simulink model "dae_example"  (R2026b)
settings: Solver=VariableStepAuto  StopTime=20  MaxStep=0.4  AbsTol=1e-3  EnableMultiTasking=on
libraries: fl_lib x9, SimscapeFluids_lib x6, nesl_utility x1
CloseFcn:
  | try,close(h1_HydrostaticTransmissionWithSecondaryControl),end
  | clear h1_HydrostaticTransmissionWithSecondaryControl
  | 
  | clear simlog_HydrostaticTransmissionWithSecondaryControl tout
  | clear logsout_HydrostaticTransmissionWithSecondaryControl
settings Model: Creator=The MathWorks, Inc.  LastModifiedBy=grouleau
settings SolverCC: AutoScaleAbsTol=off
settings DataIOCC: DSMLogging=off  LimitDataPoints=on  MaxDataPoints=10000  ReturnWorkspaceOutputs=off  SaveFormat=Array  SignalLoggingName=logsout_HydrostaticTransmissionWithSecondaryControl
settings OptimizationCC: LifeSpan=inf  MemsetInitFltsAndDblsToZero=off  ReuseModelBlockBuffer=off
settings DebuggingCC: AllowSymbolicDim=off  ArithmeticOperatorsInVariantConditions=warning  PregeneratedLibrarySubsystemCodeDiagnostic=none  SFExecutionAtInitializationDiag=none  SFNoUnconditionalDefaultTransitionDiag=warning  SFUnexpectedBacktrackingDiag=warning  SaveWithParameterizedLinksMsg=none  SignalResolutionControl=TryResolveAllWithWarning  StateNameClashWarn=warning
settings HardwareCC: ProdEndianess=Unspecified  ProdHWDeviceType=32-bit Generic  ProdIntDivRoundTo=Undefined  ProdLargestAtomicFloat=None
settings ModelReferenceCC: PropagateSignalLabelsOutOfModel=off
settings SFSimCC: CustomCodeUndefinedFunction=UseInterfaceOnly  SimUseLocalCustomCode=off
settings RTWCC: DLArmComputeVersion=19.05  RTWUseLocalCustomCode=off
settings CodeAppCC: StateflowObjectComments=on
settings GRTTargetCC: CombineOutputUpdateFcns=off  GRTInterface=on  TargetFcnLib=ansi_tfl_tmw.mat  TargetLangStandard=C89/C90 (ANSI)
settings ConfigComp: CovExternalEMLEnable=off  CovSFcnEnable=off  CovSaveCumulativeToWorkspaceVar=on  CovSaveSingleToWorkspaceVar=on
settings SimscapeCC: SimscapeLogName=simlog_HydrostaticTransmissionWithSecondaryControl  SimscapeLogSimulationStatistics=on  SimscapeLogType=all  SimscapeUseEnergyAccounting=off

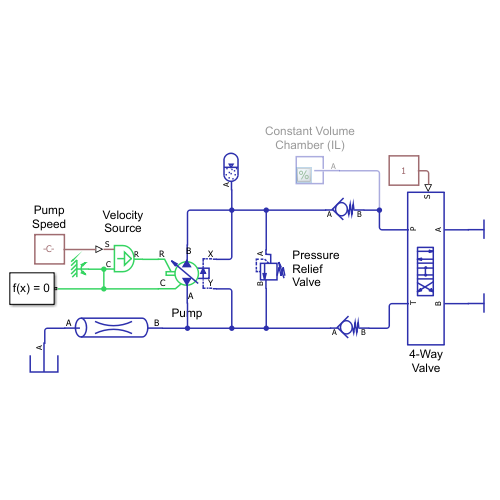
[thumbnail: Simulink's stored preview of the top-level diagram]
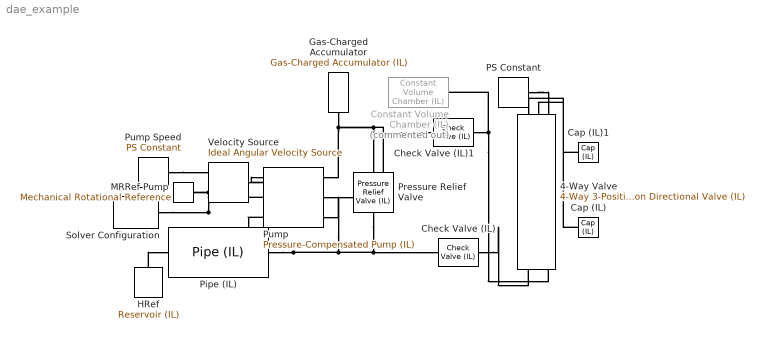
== system dae_example ==
  4-Way Valve : SimscapeFluids_lib/Isothermal Liquid/Valves & Orifices/Directional Control Valves/4-Way 3-Position Directional Valve (IL)  Tag=Factory Generic  open_orifices_pos=fluids.isothermal_liquid.valves_orifices.directional_control_valves.enum.directional_valve_open_orifices_pos_neg.PA_BT  open_orifices_neu=fluids.isothermal_liquid.valves_orifices.directional_control_valves.enum.directional_valve_open_orifices_neutral.PA_PB_AT_BT  open_orifices_neg=fluids.isothermal_liquid.valves_orifices.directional_control_valves.enum.directional_valve_open_orifices_pos_neg.PB_AT  neutral_assert_action=0  area_spec=1  valve_spec=1  del_S_max=5 mm  area_max=3.8 mm^2  del_S_TLU=[0, .00125, .0025, .00375, .005] m  valve_area_TLU="[  1e-12 4e-12 1e-05 1.02e-05 ] m^2"  del_S_vol_flow_TLU=[0, .00125, .0025, .00375, .005] m  p_diff_TLU="[  -5e+06 -2e+06 2e+06 5e+06 ] Pa"  vol_flow_TLU="[  -1e-12 -6e-14 6e+12 1e+11 ; -8e-08 -4e-08 4e+06 8e+06 ; -0.0025 -0.00103 0.001 0.0024 ; -0.00258 -0.001032 0.00106 0.00247 ; ] m^3/s"  p_diff_TLU_const=[-.1, .3, .5, .7] MPa  vol_flow_TLU_const=[-.0009, .0016, .002, .0024] m^3/s  area_const=1e-4 m^2  area_leak=1e-9 m^2  area=inf m^2  Cd=0.7  Re_c=150  smoothing_factor=0  pressure_recovery=false  S_max_PA=4.9 mm  del_S_max_PA=0.0049999 m  area_max_PA=0.5e-4 m^2  del_S_TLU_PA=[0, .00125, .0025, .00375, .005] m  valve_area_TLU_PA=[1.0e-9, 2.0352e-7, 4.0736e-5, 0.00011438, 0.00034356] m^2  del_S_vol_flow_TLU_PA=[0, .00125, .0025, .00375, .005] m  p_diff_TLU_PA=[-10000000.0, -5000000.0, -2000000.0, 2000000.0, 5000000.0, 10000000.0] Pa  vol_flow_TLU_PA=[-1.0e-7, -7.0711e-8, -4.4721e-8, 4.4721e-8, 7.0711e-8, 1.0e-7; -2.0352e-5, -1.4391e-5, -9.1017e-6, 9.1017e-6, 1.4391e-5, 2.0352e-5; -0.0040736, -0.0028805, -0.0018218, 0.0018218, 0.0028805, 0.0040736; -0.011438, -0.0080879, -0.0051152, 0.0051152, 0.0080879, 0.011438; -0.034356, -0.024293, -0.015364, 0.015364, 0.024293, 0.034356] m^3/s  area_const_PA=1e-4 m^2  p_diff_TLU_const_PA=[-.1, .3, .5, .7] MPa  vol_flow_TLU_const_PA=[-.0009, .0016, .002, .0024] m^3/s  S_max_PB=-4.9 mm  del_S_max_PB=0.0049999 m  area_max_PB=0.5e-4 m^2  del_S_TLU_PB=[0, .00125, .0025, .00375, .005] m  valve_area_TLU_PB=[1.0e-9, 2.0352e-7, 4.0736e-5, 0.00011438, 0.00034356] m^2  del_S_vol_flow_TLU_PB=[0, .00125, .0025, .00375, .005] m  p_diff_TLU_PB=[-10000000.0, -5000000.0, -2000000.0, 2000000.0, 5000000.0, 10000000.0] Pa  vol_flow_TLU_PB=[-1.0e-7, -7.0711e-8, -4.4721e-8, 4.4721e-8, 7.0711e-8, 1.0e-7; -2.0352e-5, -1.4391e-5, -9.1017e-6, 9.1017e-6, 1.4391e-5, 2.0352e-5; -0.0040736, -0.0028805, -0.0018218, 0.0018218, 0.0028805, 0.0040736; -0.011438, -0.0080879, -0.0051152, 0.0051152, 0.0080879, 0.011438; -0.034356, -0.024293, -0.015364, 0.015364, 0.024293, 0.034356] m^3/s  area_const_PB=1e-4 m^2  p_diff_TLU_const_PB=[-.1, .3, .5, .7] MPa  vol_flow_TLU_const_PB=[-.0009, .0016, .002, .0024] m^3/s  S_max_AB=7.5e-3 m  del_S_max_AB=0.005 m  area_max_AB=1e-4 m^2  del_S_TLU_AB=[0, .00125, .0025, .00375, .005] m  valve_area_TLU_AB=[1e-10, 1e-05, 4e-05, 6e-05, .0001] m^2  del_S_vol_flow_TLU_AB=[0, .00125, .0025, .00375, .005] m  p_diff_TLU_AB=[-.1, .3, .5, .7] MPa  vol_flow_TLU_AB=[-1e-08, 2.2e-08, 2.8e-08, 3.4e-08; -9e-06, .00015, .0002, .00024; -.00036, .00063, .00081, .00096; -.00054, .00094, .0012, .0014; -.00091, .0016, .002, .0024] m^3/s  area_const_AB=1e-4 m^2  p_diff_TLU_const_AB=[-.1, .3, .5, .7] MPa  vol_flow_TLU_const_AB=[-.0009, .0016, .002, .0024] m^3/s  S_max_AT=-4.9 mm  del_S_max_AT=0.0049999 m  area_max_AT=0.5e-4 m^2  del_S_TLU_AT=[0, .00125, .0025, .00375, .005] m  valve_area_TLU_AT=[1.0e-9, 2.0352e-7, 4.0736e-5, 0.00011438, 0.00034356] m^2  del_S_vol_flow_TLU_AT=[0, .00125, .0025, .00375, .005] m  p_diff_TLU_AT=[-10000000.0, -5000000.0, -2000000.0, 2000000.0, 5000000.0, 10000000.0] Pa  vol_flow_TLU_AT=[-1.0e-7, -7.0711e-8, -4.4721e-8, 4.4721e-8, 7.0711e-8, 1.0e-7; -2.0352e-5, -1.4391e-5, -9.1017e-6, 9.1017e-6, 1.4391e-5, 2.0352e-5; -0.0040736, -0.0028805, -0.0018218, 0.0018218, 0.0028805, 0.0040736; -0.011438, -0.0080879, -0.0051152, 0.0051152, 0.0080879, 0.011438; -0.034356, -0.024293, -0.015364, 0.015364, 0.024293, 0.034356] m^3/s  area_const_AT=1e-4 m^2  p_diff_TLU_const_AT=[-.1, .3, .5, .7] MPa  vol_flow_TLU_const_AT=[-.0009, .0016, .002, .0024] m^3/s  S_max_BT=4.9 mm  del_S_max_BT=0.0049999 m  area_max_BT=0.5e-4 m^2  del_S_TLU_BT=[0, .00125, .0025, .00375, .005] m  valve_area_TLU_BT=[1.0e-9, 2.0352e-7, 4.0736e-5, 0.00011438, 0.00034356] m^2  del_S_vol_flow_TLU_BT=[0, .00125, .0025, .00375, .005] m  p_diff_TLU_BT=[-10000000.0, -5000000.0, -2000000.0, 2000000.0, 5000000.0, 10000000.0] Pa  vol_flow_TLU_BT=[-1.0e-7, -7.0711e-8, -4.4721e-8, 4.4721e-8, 7.0711e-8, 1.0e-7; -2.0352e-5, -1.4391e-5, -9.1017e-6, 9.1017e-6, 1.4391e-5, 2.0352e-5; -0.0040736, -0.0028805, -0.0018218, 0.0018218, 0.0028805, 0.0040736; -0.011438, -0.0080879, -0.0051152, 0.0051152, 0.0080879, 0.011438; -0.034356, -0.024293, -0.015364, 0.015364, 0.024293, 0.034356] m^3/s  area_const_BT=1e-4 m^2  p_diff_TLU_const_BT=[-.1, .3, .5, .7] MPa  vol_flow_TLU_const_BT=[-.0009, .0016, .002, .0024] m^3/s  S_max_PT=0 m  del_S_max_PT=0.005 m  area_max_PT=1e-4 m^2  del_S_TLU_PT=[0, .00125, .0025, .00375, .005] m  valve_area_TLU_PT=[1e-10, 1e-05, 4e-05, 6e-05, .0001] m^2  del_S_vol_flow_TLU_PT=[0, .00125, .0025, .00375, .005] m  p_diff_TLU_PT=[-.1, .3, .5, .7] MPa  vol_flow_TLU_PT=[-1e-08, 2.2e-08, 2.8e-08, 3.4e-08; -9e-06, .00015, .0002, .00024; -.00036, .00063, .00081, .00096; -.00054, .00094, .0012, .0014; -.00091, .0016, .002, .0024] m^3/s
      settings: LibrarySourceBlock=SimscapeFluids_lib/Isothermal Liquid/Valves & Orifices/Directional Control Valves/4-Way 3-Position Directional Valve (IL)
  Cap (IL) : fl_lib/Isothermal Liquid/Elements/Cap (IL)  p_specify=off  p_priority=None  p=0.101325 MPa  p_nominal_specify=off  p_nominal_value=1  p_nominal_unit=MPa
  Cap (IL)1 : fl_lib/Isothermal Liquid/Elements/Cap (IL)  p_specify=off  p_priority=None  p=0.101325 MPa  p_nominal_specify=off  p_nominal_value=1  p_nominal_unit=MPa
  Check Valve (IL) : SimscapeFluids_lib/Isothermal Liquid/Valves & Orifices/Directional Control Valves/Check Valve (IL)  opening_spec=fluids.isothermal_liquid.valves_orifices.enum.PressureOpeningSpec.Linear  pressure_control_spec=fluids.isothermal_liquid.valves_orifices.enum.pressure_control_spec.dp  p_crack_differential=0.01 MPa  p_crack_gauge=0.1 MPa  press_max_differential=0.1 MPa  press_max_gauge=0.2 MPa  area_max=1e-4 m^2  area_leak=1e-10 m^2  p_diff_TLU=[0.01 : 0.01 : 0.1] MPa  valve_area_TLU=[1e-10, 1e-05, 2e-05, 3e-05, 4e-05, 5e-05, 6e-05, 7.5e-05, 8.5e-05, .0001] m^2  vol_flow_TLU=[.000358, .045, .11, .191, .284, .39, .505, .63, .764, .905] .* 1e-3 m^3/s  area=inf m^2  Cd=0.64  Re_c=150  smoothing_factor=0.01  pressure_recovery=false  opening_dynamics=false  tau=0.1 s
  Check Valve (IL)1 : SimscapeFluids_lib/Isothermal Liquid/Valves & Orifices/Directional Control Valves/Check Valve (IL)  opening_spec=fluids.isothermal_liquid.valves_orifices.enum.PressureOpeningSpec.Linear  pressure_control_spec=fluids.isothermal_liquid.valves_orifices.enum.pressure_control_spec.dp  p_crack_differential=0.01 MPa  p_crack_gauge=0.1 MPa  press_max_differential=0.1 MPa  press_max_gauge=0.2 MPa  area_max=1e-4 m^2  area_leak=1e-10 m^2  p_diff_TLU=[0.01 : 0.01 : 0.1] MPa  valve_area_TLU=[1e-10, 1e-05, 2e-05, 3e-05, 4e-05, 5e-05, 6e-05, 7.5e-05, 8.5e-05, .0001] m^2  vol_flow_TLU=[.000358, .045, .11, .191, .284, .39, .505, .63, .764, .905] .* 1e-3 m^3/s  area=inf m^2  Cd=0.64  Re_c=150  smoothing_factor=0.01  pressure_recovery=false  opening_dynamics=false  tau=0.1 s
  Constant Volume Chamber (IL) : fl_lib/Isothermal Liquid/Elements/Constant Volume Chamber (IL)  Commented=on  volume=0.001 m^3  p_I_specify=off  p_I_priority=High  p_I=0.101325 MPa  p_I_nominal_specify=off  p_I_nominal_value=1  p_I_nominal_unit=MPa
  Gas-Charged Accumulator : SimscapeFluids_lib/Isothermal Liquid/Tanks & Accumulators/Gas-Charged Accumulator (IL)  capacity=5 l  dead_volume=4e-5 m^3  p_precharge=101375 Pa  k_sh=1.4  stiff_coeff=1e10 Pa/m^3  dynamic_compressibility=simscape.enum.onoff.off  liquid_volume_specify=on  liquid_volume_priority=High  liquid_volume=0 m^3  liquid_volume_nominal_specify=off  liquid_volume_nominal_value=1  liquid_volume_nominal_unit=m^3  liquid_mass_specify=off  liquid_mass_priority=None  liquid_mass=5 kg  liquid_mass_nominal_specify=off  liquid_mass_nominal_value=1  liquid_mass_nominal_unit=kg  p_I_specify=off  p_I_priority=None  p_I=202650 Pa  p_I_nominal_specify=off  p_I_nominal_value=1  p_I_nominal_unit=Pa
      settings: LibrarySourceBlock=SimscapeFluids_lib/Isothermal Liquid/Tanks & Accumulators/Gas-Charged Accumulator (IL)
  HRef : fl_lib/Isothermal Liquid/Elements/Reservoir (IL)  Tag=Factory Generic  pressure_input=false  pressure_spec=foundation.enum.pressure_spec.atmospheric  reservoir_pressure=0.101325 MPa
  MRRef Pump : fl_lib/Mechanical/Rotational Elements/Mechanical Rotational Reference  Tag=Factory Generic
  PS Constant : fl_lib/Physical Signals/Sources/PS Constant  constant=1
  Pipe (IL) : fl_lib/Isothermal Liquid/Elements/Pipe (IL)  length=5 m  area=0.01 m^2  Dh=0.1128 m  length_add=1 m  roughness=15e-6 m  Re_lam=2000  Re_tur=4000  shape_factor=64  dynamic_compressibility=true  inertia=false  p0=0.101325 MPa  mdot0=0 kg/s
  Pressure Relief Valve : SimscapeFluids_lib/Isothermal Liquid/Valves & Orifices/Pressure Control Valves/Pressure Relief Valve (IL)  Tag=Factory Generic  set_pressure_spec=foundation.enum.constant_controlled.constant  opening_spec=1  pressure_spec=fluids.isothermal_liquid.valves_orifices.enum.pressure_control_spec.dp  p_set_gauge=0.1 MPa  p_set_differential=105 bar  p_range=5.6 bar  area_max=1e-4 m^2  area_leak=1e-8 m^2  p_diff_TLU=[30.15e5 : 15e3 : 31.35e5] Pa  p_gauge_TLU=[0.2 : 0.2 : 1.2] MPa  valve_area_TLU=[1 : 1 : 9] .* 1e-5 m^2  vol_flow_TLU=[1e-09, 3.6e-05, 8.9e-05, .00015, .00023, .00031] m^3/s  area=inf m^2  Cd=0.7  Re_c=150  smoothing_factor=0  pressure_recovery=false  opening_dynamics=0  tau=0.1 s
      settings: LibrarySourceBlock=SimscapeFluids_lib/Isothermal Liquid/Valves & Orifices/Pressure Control Valves/Pressure Relief Valve (IL)
  Pump : SimscapeFluids_lib/Isothermal Liquid/Pumps & Motors/Pressure-Compensated Pump (IL)  Tag=Factory Generic  leakage_friction_spec=fluids.isothermal_liquid.pumps_motors.enum.pump_motor_loss_spec.analytical  displacement_nominal=1.2e-4 m^3/rad  omega_nominal=188 rad/s  p_nominal=1e7 Pa  vol_eff_nominal=0.85  no_load_torque=0 N*m  p_diff_eff_TLU=[.1, 1, 2] MPa  omega_eff_TLU=[250, 500, 1000, 2000, 3000, 4000] rpm  displacement_eff_TLU=[-30, -19, 19, 30] cm^3/rev  vol_eff_TLU=repmat([.816, .908, .954, .977, .981, .984; .325, .663, .831, .916, .925, .946; .137, .568, .78, .892, .893, .91], 1, 1, 4)  mech_eff_TLU=repmat([.996, .996, .996, .996, .996, .996; .988, .989, .989, .989, .989, .99; .981, .981, .982, .982, .983, .984], 1, 1, 4)  p_diff_loss_TLU=[.1, 1, 2] MPa  omega_loss_TLU=[250, 500, 1000, 2000, 3000, 4000] rpm  vol_loss_TLU=repmat(1e-3 * [.023, .023, .023, .023, .0285, .032; .0844, .0842, .0845, .084, .1125, .108; .1079, .108, .11, .108, .1605, .18], 1, 1, 4) m^3/s  mech_loss_TLU=repmat([.002, .002, .002, .002, .002, .002; .0607, .0556, .0556, .0556, .0556, .0505; .1937, .1937, .1833, .1833, .1729, .1626], 1, 1, 4) N*m  vol_eff_min=1e-3  vol_eff_max=1  mech_eff_min=1e-3  mech_eff_max=1  pressure_threshold=1e-3 MPa  omega_threshold=100 rpm  supplied_range_check=simscape.enum.assert.action.none  pump_mode_check=simscape.enum.assert.action.none  pressure_check=simscape.enum.assert.action.none  mech_eff_nominal=0.88  displacement_loss_TLU=[-30, -19, 19, 30] cm^3/rev  displacement_max=1.2e-4 m^3/rad  displacement_min=0.1 cm^3/rev  p_set_differential=1e7 Pa  p_range=6e5 Pa  smoothing_factor=0  displacement_dynamics=false  tau=0.1 s  p_min_valid=0.101325 MPa
      settings: LibrarySourceBlock=SimscapeFluids_lib/Isothermal Liquid/Pumps & Motors/Pressure-Compensated Pump (IL)
  Pump Speed : fl_lib/Physical Signals/Sources/PS Constant  constant=1770/60*2*pi rad/s
  Solver Configuration : nesl_utility/Solver Configuration  PhysicalDomain=network_engine_domain  SubClassName=solver  LeftPortType=input  RightPortType=generic  Tones=[]  Harmonics=[]  SimulateNoise=off  Profile=off  UseLocalSampling=off  EnableSwitchedLinearOptims=on  FrequencyDomain=off  UseCCode=off  RelTol=0.001  AbsTol=1e-06  MinStep=1e-09  ToWorkspace=off  RevertToSquareIcSolve=off  NumHomotopyIterations=100  PhasorMode=off  PhasorModeNumHarmonics=1  ConsistencySolver=NEWTON_XTOL_AFTER_FTOL  CanonicalOrdering=UNORDERED  OptimizeIntermediates=UNOPTIMIZED  MulticoreSolverChoice=BACKWARD_EULER  IndexReductionMethod=DerivativeReplacement  DoDC=off  ResidualTolerance=1e-9  ConsistencyTolSource=GLOBAL  ConsistencyAbsTol=0.001  ConsistencyRelTol=0.001  ConsistencyTolFactor=0.001  UseLocalSolver=off  LocalSolverChoice=NE_BACKWARD_EULER_ADVANCER  ResolveIndetEquations=on  FunctionEvalNumThread=1  LocalSolverSampleTime=.001  DoFixedCost=off  MaxNonlinIter=3  MaxModeIter=2  ComputeImpulses=off  ImpulseIterations=2  LinearAlgebra=auto  LinearAlgebraNumThread=0  EquationFormulation=NE_TIME_EF  DelaysMemoryBudget=1024  AutomaticFiltering=on  FilteringTimeConstant=0.001  PartitionStorageMethod=AS_NEEDED  PartitionMemoryBudget=1024  PartitionMethod=FAST  MultibodyUseLocalSolver=off  MultibodyLocalSolverChoice=ODE1  MultibodyLocalSolverSampleTime=0.001
  Velocity Source : fl_lib/Mechanical/Mechanical Sources/Ideal Angular Velocity Source  Tag=Factory Generic
  connections:
  Velocity Source/RConn2 -- Solver Configuration/RConn1 -- Pump/RConn2 -- MRRef Pump/LConn1
  Pump Speed/RConn1 -- Velocity Source/RConn1
  Velocity Source/LConn1 -- Pump/RConn1
  Pump/LConn1 -- Check Valve (IL)1/LConn1 -- Pressure Relief Valve/LConn1 -- Pump/LConn3 -- Gas-Charged Accumulator/RConn1
  Pressure Relief Valve/RConn1 -- Pump/LConn2 -- Pump/RConn3 -- Pipe (IL)/RConn1 -- Check Valve (IL)/LConn1
  Cap (IL)1/LConn1 -- 4-Way Valve/LConn2
  Cap (IL)/LConn1 -- 4-Way Valve/LConn3
  PS Constant/RConn1 -- 4-Way Valve/LConn1
  Check Valve (IL)1/RConn1 -- Constant Volume Chamber (IL)/LConn1 -- 4-Way Valve/RConn1
  Check Valve (IL)/RConn1 -- 4-Way Valve/RConn2
  HRef/LConn1 -- Pipe (IL)/LConn1
